simulink model "codeur_hamming"  (R2023b)
settings: Solver=FixedStepDiscrete  StartTime=0.0  StopTime=112  FixedStep=1  RelTol=1e-3
settings Model: Creator=e2507457  LastModifiedBy=e2507457

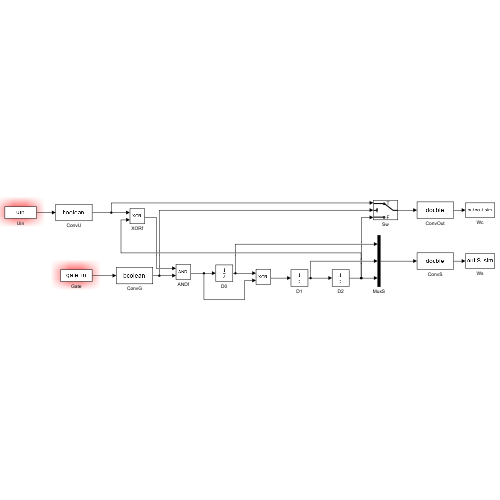
[thumbnail: Simulink's stored preview of the top-level diagram]
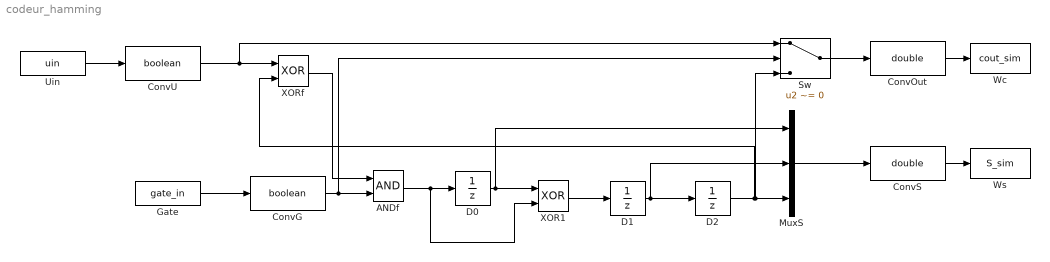
== system codeur_hamming ==
  ANDf : Logic  AllPortsSameDT=off  OutDataTypeStr=boolean
  ConvG : DataTypeConversion  OutDataTypeStr=boolean  SaturateOnIntegerOverflow=off  RndMeth=Floor
  ConvOut : DataTypeConversion  OutDataTypeStr=double  SaturateOnIntegerOverflow=off  RndMeth=Floor
  ConvS : DataTypeConversion  OutDataTypeStr=double  SaturateOnIntegerOverflow=off  RndMeth=Floor
  ConvU : DataTypeConversion  OutDataTypeStr=boolean  SaturateOnIntegerOverflow=off  RndMeth=Floor
  D0 : UnitDelay  HasFrameUpgradeWarning=on
  D1 : UnitDelay  HasFrameUpgradeWarning=on
  D2 : UnitDelay  HasFrameUpgradeWarning=on
  Gate : FromWorkspace  VariableName=gate_in  SampleTime=1  Interpolate=off  OutputAfterFinalValue=Holding final value
  MuxS : Mux  Inputs=3
  Sw : Switch  Criteria=u2 ~= 0  SaturateOnIntegerOverflow=off  InputSameDT=off
  Uin : FromWorkspace  VariableName=uin  SampleTime=1  Interpolate=off  OutputAfterFinalValue=Holding final value
  Wc : ToWorkspace  VariableName=cout_sim  SampleTime=-1
  Ws : ToWorkspace  VariableName=S_sim  SampleTime=-1
  XOR1 : Logic  Operator=XOR  AllPortsSameDT=off  OutDataTypeStr=boolean
  XORf : Logic  Operator=XOR  AllPortsSameDT=off  OutDataTypeStr=boolean
  wires:
  XORf/1 -> ANDf/1
  Uin/1 -> ConvU/1
  ConvU/1 -> Sw/1, XORf/1
  Gate/1 -> ConvG/1
  ConvG/1 -> ANDf/2, Sw/2
  ANDf/1 -> XOR1/2, D0/1
  D0/1 -> MuxS/1, XOR1/1
  XOR1/1 -> D1/1
  D1/1 -> D2/1, MuxS/2
  D2/1 -> Sw/3, MuxS/3, XORf/2
  Sw/1 -> ConvOut/1
  ConvS/1 -> Ws/1
  MuxS/1 -> ConvS/1
  ConvOut/1 -> Wc/1
